simulink model "fw_telemetry"  (R2026b)
settings: Solver=VariableStepAuto
undefined symbols (not defined in the file or in its folder): Ts
settings Model: Creator=aomar  LastModifiedBy=aomar

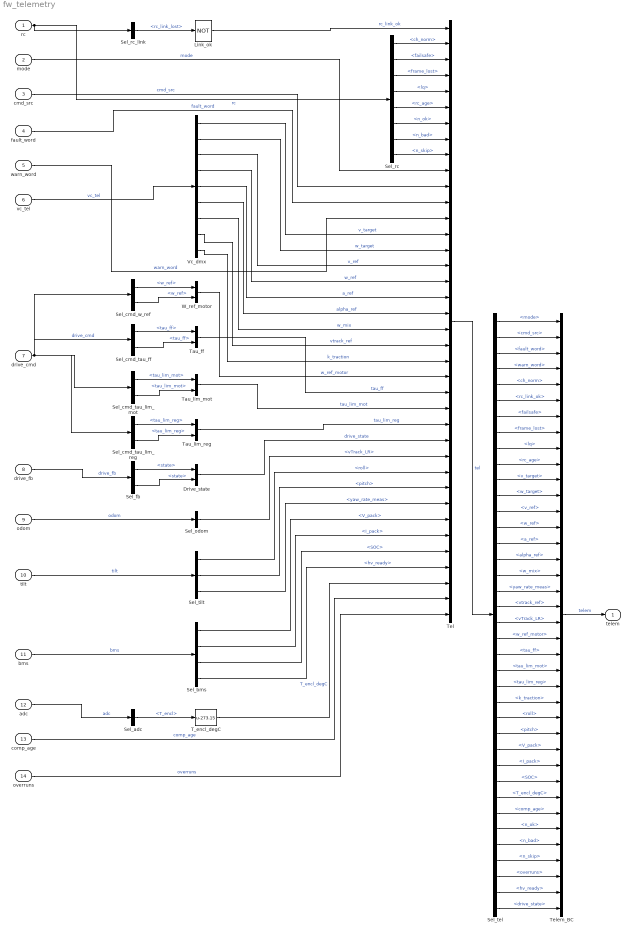
== system fw_telemetry ==
  rc : Inport  SampleTime=Ts.ctrl
  mode : Inport  Port=2  OutDataTypeStr=uint8  SampleTime=Ts.ctrl
  cmd_src : Inport  Port=3  OutDataTypeStr=uint8  SampleTime=Ts.ctrl
  fault_word : Inport  Port=4  OutDataTypeStr=uint32  SampleTime=Ts.ctrl
  warn_word : Inport  Port=5  OutDataTypeStr=uint32  SampleTime=Ts.ctrl
  vc_tel : Inport  Port=6  OutDataTypeStr=single  PortDimensions=11  SampleTime=Ts.ctrl
  drive_cmd : Inport  Port=7  OutDataTypeStr=Bus: Bus_DriveCmd  SampleTime=Ts.ctrl
  drive_fb : Inport  Port=8  OutDataTypeStr=Bus: Bus_DriveFb  SampleTime=Ts.ctrl
  odom : Inport  Port=9  OutDataTypeStr=Bus: Bus_OdomMeas  SampleTime=Ts.ctrl
  tilt : Inport  Port=10  SampleTime=Ts.ctrl
  bms : Inport  Port=11  OutDataTypeStr=Bus: Bus_BmsStatus  SampleTime=Ts.ctrl
  adc : Inport  Port=12  SampleTime=Ts.ctrl
  comp_age : Inport  Port=13  OutDataTypeStr=single  SampleTime=Ts.ctrl
  overruns : Inport  Port=14  OutDataTypeStr=uint32  SampleTime=Ts.ctrl
  Drive_state : Concatenate
  Link_ok : Logic  Operator=NOT  Inputs=1  AllPortsSameDT=off  OutDataTypeStr=boolean
  Sel_adc : BusSelector  OutputSignals=T_encl
  Sel_bms : BusSelector  OutputSignals=V_pack,I_pack,SOC,hv_ready
  Sel_cmd_tau_ff : BusSelector  OutputSignals=L.tau_ff,R.tau_ff
  Sel_cmd_tau_lim_mot : BusSelector  OutputSignals=L.tau_lim_mot,R.tau_lim_mot
  Sel_cmd_tau_lim_reg : BusSelector  OutputSignals=L.tau_lim_reg,R.tau_lim_reg
  Sel_cmd_w_ref : BusSelector  OutputSignals=L.w_ref,R.w_ref
  Sel_fb : BusSelector  OutputSignals=L.state,R.state
  Sel_odom : BusSelector  OutputSignals=vTrack_LR
  Sel_rc : BusSelector  OutputSignals=ch_norm,failsafe,frame_lost,lq,rc_age,n_ok,n_bad,n_skip
  Sel_rc_link : BusSelector  OutputSignals=rc_link_lost
  Sel_tel : BusSelector  OutputSignals=mode,cmd_src,fault_word,warn_word,ch_norm,rc_link_ok,failsafe,frame_lost,lq,rc_age,v_target,w_target,v_ref,w_ref,a_ref,alpha_ref,w_mix,yaw_rate_meas,vtrack_ref,vTrack_LR,w_ref_motor,tau_ff,tau_lim_mot,tau_lim_reg,k_traction,roll,pitch,V_pack,I_pack,SOC,T_encl_degC,comp_age,n_ok,n_bad,n_skip,overruns,hv_ready,drive_state
  Sel_tilt : BusSelector  OutputSignals=roll,pitch,yaw_rate_meas
  T_encl_degC : Bias  Bias=-273.15  SaturateOnIntegerOverflow=off
  Tau_ff : Concatenate
  Tau_lim_mot : Concatenate
  Tau_lim_reg : Concatenate
  Tel : BusCreator  Inputs=38
  Telem_BC : BusCreator  Inputs=38  OutDataTypeStr=Bus: Bus_FwTelemetry  NonVirtualBus=on
      settings: InheritFromInputs=off
  Vc_dmx : Demux  Outputs=[1 1 1 1 1 1 1 2 2]
  W_ref_motor : Concatenate
  telem : Outport  OutDataTypeStr=Bus: Bus_FwTelemetry
  wires:
  rc/1 -> Sel_rc/1, Sel_rc_link/1  "rc"
  mode/1 -> Tel/10  "mode"
  cmd_src/1 -> Tel/11  "cmd_src"
  fault_word/1 -> Tel/12  "fault_word"
  warn_word/1 -> Tel/13  "warn_word"
  vc_tel/1 -> Vc_dmx/1  "vc_tel"
  drive_cmd/1 -> Sel_cmd_tau_lim_reg/1, Sel_cmd_w_ref/1, Sel_cmd_tau_lim_mot/1, Sel_cmd_tau_ff/1  "drive_cmd"
  drive_fb/1 -> Sel_fb/1  "drive_fb"
  odom/1 -> Sel_odom/1  "odom"
  tilt/1 -> Sel_tilt/1  "tilt"
  bms/1 -> Sel_bms/1  "bms"
  adc/1 -> Sel_adc/1  "adc"
  comp_age/1 -> Tel/37  "comp_age"
  overruns/1 -> Tel/38  "overruns"
  Sel_rc_link/1 -> Link_ok/1  "<rc_link_lost>"
  Sel_cmd_w_ref/1 -> W_ref_motor/1  "<w_ref>"
  Sel_cmd_w_ref/2 -> W_ref_motor/2  "<w_ref>"
  Sel_cmd_tau_ff/1 -> Tau_ff/1  "<tau_ff>"
  Sel_cmd_tau_ff/2 -> Tau_ff/2  "<tau_ff>"
  Sel_cmd_tau_lim_mot/1 -> Tau_lim_mot/1  "<tau_lim_mot>"
  Sel_cmd_tau_lim_mot/2 -> Tau_lim_mot/2  "<tau_lim_mot>"
  Sel_cmd_tau_lim_reg/1 -> Tau_lim_reg/1  "<tau_lim_reg>"
  Sel_cmd_tau_lim_reg/2 -> Tau_lim_reg/2  "<tau_lim_reg>"
  Sel_fb/1 -> Drive_state/1  "<state>"
  Sel_fb/2 -> Drive_state/2  "<state>"
  Sel_adc/1 -> T_encl_degC/1  "<T_encl>"
  Vc_dmx/1 -> Tel/14  "v_target"
  Vc_dmx/2 -> Tel/15  "w_target"
  Vc_dmx/3 -> Tel/16  "v_ref"
  Vc_dmx/4 -> Tel/17  "w_ref"
  Vc_dmx/5 -> Tel/18  "a_ref"
  Vc_dmx/6 -> Tel/19  "alpha_ref"
  Vc_dmx/7 -> Tel/20  "w_mix"
  Vc_dmx/8 -> Tel/21  "vtrack_ref"
  Vc_dmx/9 -> Tel/22  "k_traction"
  W_ref_motor/1 -> Tel/23  "w_ref_motor"
  Tau_ff/1 -> Tel/24  "tau_ff"
  Tau_lim_mot/1 -> Tel/25  "tau_lim_mot"
  Tau_lim_reg/1 -> Tel/26  "tau_lim_reg"
  Drive_state/1 -> Tel/27  "drive_state"
  Sel_odom/1 -> Tel/28  "<vTrack_LR>"
  Sel_tilt/1 -> Tel/29  "<roll>"
  Sel_tilt/2 -> Tel/30  "<pitch>"
  Sel_tilt/3 -> Tel/31  "<yaw_rate_meas>"
  Sel_bms/1 -> Tel/32  "<V_pack>"
  Sel_bms/2 -> Tel/33  "<I_pack>"
  Sel_bms/3 -> Tel/34  "<SOC>"
  Sel_bms/4 -> Tel/35  "<hv_ready>"
  Link_ok/1 -> Tel/1  "rc_link_ok"
  T_encl_degC/1 -> Tel/36  "T_encl_degC"
  Sel_rc/1 -> Tel/2  "<ch_norm>"
  Sel_rc/2 -> Tel/3  "<failsafe>"
  Sel_rc/3 -> Tel/4  "<frame_lost>"
  Sel_rc/4 -> Tel/5  "<lq>"
  Sel_rc/5 -> Tel/6  "<rc_age>"
  Sel_rc/6 -> Tel/7  "<n_ok>"
  Sel_rc/7 -> Tel/8  "<n_bad>"
  Sel_rc/8 -> Tel/9  "<n_skip>"
  Tel/1 -> Sel_tel/1  "tel"
  Sel_tel/1 -> Telem_BC/1  "<mode>"
  Sel_tel/2 -> Telem_BC/2  "<cmd_src>"
  Sel_tel/3 -> Telem_BC/3  "<fault_word>"
  Sel_tel/4 -> Telem_BC/4  "<warn_word>"
  Sel_tel/5 -> Telem_BC/5  "<ch_norm>"
  Sel_tel/6 -> Telem_BC/6  "<rc_link_ok>"
  Sel_tel/7 -> Telem_BC/7  "<failsafe>"
  Sel_tel/8 -> Telem_BC/8  "<frame_lost>"
  Sel_tel/9 -> Telem_BC/9  "<lq>"
  Sel_tel/10 -> Telem_BC/10  "<rc_age>"
  Sel_tel/11 -> Telem_BC/11  "<v_target>"
  Sel_tel/12 -> Telem_BC/12  "<w_target>"
  Sel_tel/13 -> Telem_BC/13  "<v_ref>"
  Sel_tel/14 -> Telem_BC/14  "<w_ref>"
  Sel_tel/15 -> Telem_BC/15  "<a_ref>"
  Sel_tel/16 -> Telem_BC/16  "<alpha_ref>"
  Sel_tel/17 -> Telem_BC/17  "<w_mix>"
  Sel_tel/18 -> Telem_BC/18  "<yaw_rate_meas>"
  Sel_tel/19 -> Telem_BC/19  "<vtrack_ref>"
  Sel_tel/20 -> Telem_BC/20  "<vTrack_LR>"
  Sel_tel/21 -> Telem_BC/21  "<w_ref_motor>"
  Sel_tel/22 -> Telem_BC/22  "<tau_ff>"
  Sel_tel/23 -> Telem_BC/23  "<tau_lim_mot>"
  Sel_tel/24 -> Telem_BC/24  "<tau_lim_reg>"
  Sel_tel/25 -> Telem_BC/25  "<k_traction>"
  Sel_tel/26 -> Telem_BC/26  "<roll>"
  Sel_tel/27 -> Telem_BC/27  "<pitch>"
  Sel_tel/28 -> Telem_BC/28  "<V_pack>"
  Sel_tel/29 -> Telem_BC/29  "<I_pack>"
  Sel_tel/30 -> Telem_BC/30  "<SOC>"
  Sel_tel/31 -> Telem_BC/31  "<T_encl_degC>"
  Sel_tel/32 -> Telem_BC/32  "<comp_age>"
  Sel_tel/33 -> Telem_BC/33  "<n_ok>"
  Sel_tel/34 -> Telem_BC/34  "<n_bad>"
  Sel_tel/35 -> Telem_BC/35  "<n_skip>"
  Sel_tel/36 -> Telem_BC/36  "<overruns>"
  Sel_tel/37 -> Telem_BC/37  "<hv_ready>"
  Sel_tel/38 -> Telem_BC/38  "<drive_state>"
  Telem_BC/1 -> telem/1  "telem"
